simulink model "Sample_task_test"  (Simulink 8.1)
settings: Solver=ode4  SolverMode=SingleTasking  StartTime=0.0  StopTime=inf  FixedStep=0.0005  RelTol=1e-3
StartFcn:
  |  warndlg('Dexterit-E models cannot run under simulation. Please compile your model and run it from within Dexterit-E.');set_param(bdroot,'SimulationCommand','stop')
undefined symbols (not defined in the file or in its folder): slselsubs
libraries: simulink x4, General x3, KINARM_loads x2, KINARM_IO x1, KINARM_EP_loads x1, KINARM_general x1, Video x1, xpclib x1
(part 3 of 3)

== matlab function Trajectory subsystem/Create_Trajectory/get_arm_info ==
  settings: fimath=|
      | fimath(...
      | 'RoundMode', 'floor',...
      | 'OverflowMode', 'wrap',...
      | 'ProductMode', 'KeepLSB', 'ProductWordLength', 32,...
      | 'SumMode', 'KeepLSB', 'SumWordLength', 32,...
      | 'CastBeforeSum', false)
  data: position output double; task_status output double; use_dom_hand input double; kinarm_data input double; run_status input double; scaling input double; robot_enabled output double
function [position, task_status, robot_enabled]  = fcn(use_dom_hand, kinarm_data, run_status, scaling)
%
% get current hand position and robot enabled status
%
% May 2009
%

hpx_index = 23;
hpy_index = 24;
robot_disabled_index = 37;

%determine which arm to apply the load to
dominant_hand=kinarm_data(3,1);						%kinarm_data(3,1) tells which arm is the dominant arm
if use_dom_hand == 1
	feedback_arm = dominant_hand;
else
	feedback_arm = 3 - dominant_hand;
end

hpx = kinarm_data( feedback_arm, hpx_index );
hpy = kinarm_data( feedback_arm, hpy_index );
position = [hpx hpy];

if kinarm_data( feedback_arm, robot_disabled_index ) == 0;
    robot_enabled = 1;
else
    robot_enabled = 0;
end

% if the task has stopped/paused (i.e. run_status == 0) AND the torques outputs
% have scaled down to 0, then set the task_status = 0.
if run_status == 0 && scaling(feedback_arm) == 0
    task_status = 0;
else
    task_status = 1;
end

== matlab function Trajectory subsystem/KINARM_EP_Position_Controller/FF_FB_Position_Controller ==
  settings: fimath=|
      | fimath(...
      | 'RoundMode', 'floor',...
      | 'OverflowMode', 'wrap',...
      | 'ProductMode', 'KeepLSB', 'ProductWordLength', 32,...
      | 'SumMode', 'KeepLSB', 'SumWordLength', 32,...
      | 'CastBeforeSum', false)
  data: Force_FB output double; use_dom_hand input double; kinarm_data input double; setpoint_angles input double; setpoint_vel input double; setpoint_acc input double; Force_FF output double; Secondary_Encoders_Used input double; inertia_option_for_FF input double; primary_encoder_data input double; gain_choice input double; ForceOn input double
function [Force_FB, Force_FF] = fcn(use_dom_hand, kinarm_data, setpoint_angles, setpoint_vel, setpoint_acc, Secondary_Encoders_Used, inertia_option_for_FF, primary_encoder_data, gain_choice, ForceOn)
% This block supports the Embedded MATLAB subset.
% See the help menu for details. 
% set point is joint angles in global coordinates

% inertia_option_for_FF sets the options for which inertias to include for 
% the feed-forward model
%	0 - none
%	1 - KINARM robot only

% gain_choice sets the options for which proportional gains to use for the
% controller (does not affect the gains when secondary encoders are used)
%	1 - Standard Movement  == Highest stiffness. For primary encoders only, this is quite underdamped.
%	2 - Step Response == Reduced overshoot for primary encoders only, and lower stiffness.  Same as above for secondary encoders.

%{
L1_index = 1;				% L1 (m)
L2_index = 2;				% L2(m)
ORIENT_index = 6;			% 1=right	2=left
L1Ang_index = 17;			% L1 angle
L2Ang_index = 18;			% L2 Angle
L1Vel_index = 19;			% L1 angle
L2Vel_index = 20;			% L2 Angle

Force_FF = [0 0 0 0];
Force_FB = [0 0 0 0];
%}

%determine which arm to apply the load to
dominant_hand=kinarm_data(3,1);						%kinarm_data(3,1) tells which arm is the dominant arm
if use_dom_hand==1
	arm=dominant_hand;
else
	arm=3-dominant_hand;
end

%{

L1 = kinarm_data( arm, L1_index );
L2 = kinarm_data( arm, L2_index );
L1Ang = kinarm_data( arm, L1Ang_index );
L2Ang = kinarm_data( arm, L2Ang_index );
L1Vel = kinarm_data( arm, L1Vel_index );
L2Vel = kinarm_data( arm, L2Vel_index );
theta=[L1Ang; L2Ang];
thetavel=[L1Vel; L2Vel];
theta_primary = primary_encoder_data(arm, 1:2)';
thetavel_primary = primary_encoder_data(arm, 3:4)';

% Proportional Gain
if gain_choice == 1         %If the "standard movement" gain choice is selected:
    Kp = [200 0; 0 200];	%proportional gain for KINARM EP robot, primary encoders only - high stiffness
else
    Kp = [85 0; 0 85];		%proportional gain for KINARM EP robot, primary encoders only - reduced overshoot
end
Kp_1 = [0 0; 0 0];			%proportional gain for KINARM EP robot, primary encoders if used in conjunction with secondary
Kp_2 = [1 0; 0 1];		%proportional gain for KINARM EP robot, secondary encoders if used in conjunction with primary

% Derivative gain
Kv = [3.5 0; 0 3.5];		% Derivative gain for KINARM EP robot, primary encoders only				
Kv_1 = [2.5 0; 0 2.5];		% Derivative gain for KINARM EP robot, primary encoders if used in conjunction with secondary
Kv_2 = [6 0; 0 6];          % Derivative gain for KINARM EP robot, secondary encoders if used in conjunction with primary	



error = setpoint_angles - theta;
error_vel = setpoint_vel - thetavel;

error_primary = setpoint_angles - theta_primary;
error_vel_primary = setpoint_vel - thetavel_primary;

% THE FOLLOWING ARE TYPICAL VALUES FOR THE KINARM End Point robot (Rev1)
I1_prox		= 0.018;			%inertia of KINARM segment 1, kg-m^2 at shoulder
I2_5_prox	= 0.034;			%inertia of KINARM segments 2&5, kg-m^2 at elbow
I3_prox		= 0.014;			%inertia of KINARM segment 3, kg-m^2 at elbow
I4_prox		= 0.022;			%inertia of KINARM segment 4, kg-m^2 at shoulder
Im1 = 0.0047;			%inertia of motor 1, after 6x gear ratio, kg-m^2
Im2 = 0.0047;			%inertia of motor 2, after 6x gear ratio, kg-m^2
M2 = 0.62;				%mass of KINARM segment2 and 5 (kg)
M4 = 0.80;				%mass of segment 4 (kg)
L3 = 0.187;				%crank length (m)
delta = 0;				%0 degrees, angle between segments 2 and 5
x2 = 0.20;				%center of mass of segments 2+5 (m)
x4 = 0.12;				%center of mass of segment 4 (m)



theta2_1 = setpoint_angles(2) - setpoint_angles(1);
sin21 = sin(theta2_1);
cos21 = cos(theta2_1);
sin51 = sin(theta2_1 - delta);
cos51 = cos(theta2_1 - delta);

% The following equations implement the equations of motion for the KINARM robot
% For simplicity, we have ignored the off-axis components of inertia due to their
% negligible contributions
A = I1_prox + I4_prox + Im1 + M2*L1^2;
B = M2*L1*(x2*cos21) + M4*L3*(x4*cos51);
D = I2_5_prox + I3_prox + Im2 + M4*L3^2;
C = M2*L1*(x2*sin21) + M4*L3*(x4*sin51);

M = [A B; B D];	%inertial matrix
CC = [0 -C; C 0] * diag(setpoint_vel);	%coriolis and centripetal forces

if inertia_option_for_FF == 0;			%no feed-forward control
	TRQ_FF = [0; 0];
else
	TRQ_FF = M*setpoint_acc + CC*setpoint_vel;
end

if Secondary_Encoders_Used(arm) == 0
	% Only use primary encoder feedback
	TRQ_FB = Kp*error + Kv*error_vel;
else
	% Use both primary and secondary encoders - note: secondary encoder information under these conditions is contained error and error_vel
	TRQ_FB = Kp_2*error + Kv_2*error_vel + Kp_1*error_primary + Kv_1*error_vel_primary;
end

%convert torques (applied to links) to forces (applied at end-point);
A1 = -L1*sin(L1Ang);
A2 = L1*cos(L1Ang);
A3 = -L2*sin(L2Ang);
A4 = L2*cos(L2Ang);

F_FF = [A1 A2; A3 A4] \ TRQ_FF;
F_FB = [A1 A2; A3 A4] \ TRQ_FB;
%}

%%%%%%%%%%%%%%%%%%%%%%%%%%%%%%%%%%%%%%%%%%%%%%%%%%%%%%%%%%%%%%%%%%%%%%%%%%%
xPos = kinarm_data(arm,23);
yPos = kinarm_data(arm,24);
xVel = kinarm_data(arm,25);
yVel = kinarm_data(arm,26);



% FINAL FORCE CHECK
if ForceOn==1
    % Send force
    F_FB = [0; 0]; % SET WHEN EVERYTHING IS OKAY
    %F_FB = [0; 0]; % do not send force yet
else
    % No force
    F_FB = [0; 0];
end
F_FF = [0; 0];

%%%%%%%%%%%%%%%%%%%%%%%%%%%%%%%%%%%%%%%%%%%%%%%%%%%%%%%%%%%%%%%%%%%%%%%%%%%


% Flatten any bad values to 0.
if F_FF(1) ~= F_FF(1)
    F_FF(1) = 0;
end

if F_FF(2) ~= F_FF(2)
    F_FF(2) = 0;
end

if F_FB(1) ~= F_FB(1)
    F_FB(1) = 0;
end

if F_FB(2) ~= F_FB(2)
    F_FB(2) = 0;
end

%apply the forces to the correct arm 
if arm==1
	Force_FF = [F_FF' 0 0];
	Force_FB = [F_FB' 0 0];
else
	Force_FF = [0 0 F_FF'];
	Force_FB = [0 0 F_FB'];
end

== matlab function Trajectory subsystem/KINARM_EP_Position_Controller/Get_kinematics_EP/xy_to_segment_angles_EP ==
  settings: fimath=|
      | fimath(...
      | 'RoundMode', 'floor',...
      | 'OverflowMode', 'wrap',...
      | 'ProductMode', 'KeepLSB', 'ProductWordLength', 32,...
      | 'SumMode', 'KeepLSB', 'SumWordLength', 32,...
      | 'CastBeforeSum', false)
  data: use_dom_hand input double; kinarm_data input double; u input double; SEGMENT_ANG output double; robot_calib input double
function SEGMENT_ANG  = fcn(use_dom_hand, kinarm_data, u, robot_calib)

% This function converts an endpoint finger-tip position or local joint angle (shoulder, elbow) 
% to (L1Ang, L2Ang) angles for a KINARM robot where L1Ang and L2Ang are the global angles of L1 and L2  
% Note: these equations were taken from a source which defined theta1 as the global angle of L1 (i.e. theta1 = L1Ang
% and L2_L1Ang = local angle of L2 WRT L1 (but always in a R.H. coordinate frame).  So L2_L1Ang = L2Ang - L1Ang.
% Also note that we need to correct for L2_ptr

% angles_or_XY sets the options for which coordinate system to use
%	1 - (x, y) coordinates
%	2 - local coordinate joint angles (shoulder, elbow)

% NEED TO GET SHOULDER AND ELBOW ANGLE OFFSETS FROM CALIBRATION WHEN THESE BECOME AVAILABLE.
% For the KINARM End-Point robot I have assumed certain values, which will hold unless the robot
% is mounted at an angle relative to global.
% Need to decide how to deal with this for the Exoskeleton lab.

L1_index = 1;				% L1 (m)
L2_index = 2;				% L2(m)
L2ptr_index = 3;			% L2ptr(m)
SHO_ORIGIN_X_index = 4;		% shoulder origin, x position
SHO_ORIGIN_Y_index = 5;		% shoulder origin, y position
ORIENT_index = 6;			% 1=right	2=left


%determine which arm to apply the load to
dominant_hand=kinarm_data(3,1);						%kinarm_data(3,1) tells which arm is the dominant arm
if use_dom_hand==1
	arm=dominant_hand;
else
	arm=3-dominant_hand;
end

ORIENTATION = kinarm_data( arm, ORIENT_index);

% To be consistent with the Exoskeleton, the shoulder and elbow angles are stored in a 
% 'local' coordinate frame from the robot's perspective.  The right End-Point robot is 
% constructed the same a left KINARM Exoskeleton and vice-versa.  So the 'local' coordinate
% frame for a R.H. KINARM EP robot is actually a left-handed coordinate frame.
Sho_offset = robot_calib(1, arm);		% value stored in calibration in a 'local' coordinate frame.

position=[0,0];	%initialization
if length(u)==2	%input is assumed to be (x,y) position, global coordinates, (m)
    if size(u,1) == 1;
        position=u;
    else
        position=u';
    end
else			%input is assumed to be a VCODE
    position(1)=u(3);
    position(2)=u(4);
end


% calculate theta from (x,y)
L1 = kinarm_data( arm, L1_index );
L2 = kinarm_data( arm, L2_index );
L2ptr = kinarm_data( arm, L2ptr_index );
SHO_ORIGIN_X = kinarm_data( arm, SHO_ORIGIN_X_index );
SHO_ORIGIN_Y = kinarm_data( arm, SHO_ORIGIN_Y_index );

x = position(1) - SHO_ORIGIN_X;
y = position(2) - SHO_ORIGIN_Y;

L2_temp = sqrt(L2^2 + L2ptr^2);
L2_ptr_angle_shift = atan2(L2ptr, L2);			%

% The following calculation assumes that the (local) elbow angle is 
% never less than 0 (i.e. L2_L1Ang > 0 for right-handed Exoskeleton, or LEFT-HANDED End-Point, and 
% L2_L1Ang < 0 for  left-handed Exoskelton or RIGHT-HANDED End-Point).  These are always true if L2ptr > 0.  
% If L2ptr < 0, then two solutions exist, however, the one with (local) 
% elbow_angle > 0 is chosen.  
% In addition, temp is limited to +-1 to avoid an error using acos.  
% Originally this was simple clipping, but the infinite slope at acos(1)
% created instability problems, so tanh(temp + temp^3/3...) was added to 
% smooth out the transition.  The difference in angle is < 1 degree with 
% elbow angle > 30 degrees.  As the elbow extends further, the 'error' 
% is <20 degrees when full extension should theoretically happen.  For 
% L1 = 0.3m and L2 = 0.4m, the end-point error with an input point
% that in theory requires full extension is <1cm.  This end-point error
% is < 1mm when the desired endpoint is >66cm out.
% Note: tanh(temp + temp^3/3...) provides a sharper transition than 
% tanh(temp), which in turn provides a shaper one than atan(temp)
% The more terms in the tanh(temp...) series, the greater the cutoff
temp = (x^2 + y^2 - L1^2 - L2_temp^2) / (2*L1*L2_temp);
% 	temp = sign(temp) * min(abs(temp), 1);          %Not used to avoid infinite slope issue for subsequent acos
temp = tanh(temp + temp^3/3 + temp^5/5 + temp^7/7 + temp^9/9 + temp^11/11);
L2_L1Ang = acos( temp );

% if ORIENTATION == 2 %left-handed KINARM Exoskeleton 
if ORIENTATION == 1 %right-handed KINARM End-Point robot
    L2_L1Ang = -L2_L1Ang;
    L2_ptr_angle_shift = -L2_ptr_angle_shift;
end
sint = sin(L2_L1Ang);
cost = cos(L2_L1Ang);
L1Ang = atan2( ( -x*L2_temp*sint + y *(L1 + L2_temp*cost) ) , ( y*L2_temp*sint + x *(L1 + L2_temp*cost) ) );

% Likewise, there are multiple solutions for the inverse kinematics for 
% L1Ang as well. We know (based on possible arm configurations) which is 
% the correct solution for right-handed versus left-handed KINARMs.
% Sho_offset is in local coordinates.  It is translated to global as  
% L1_offset.  For "left" robots (i.e. left Exo and right EP), 
% L1Ang = -ShoAng + pi.  
% For the KINARM End-Point robot, working from the calibration 
% position (i.e. when L1Ang = L1_Offset), we know that the L1 link cannot 
% point directly backwards into the K-box.  Which for the left KINARM EP is 
% a rotation of -3/4pi or +5/4pi and for the right it is -5/4pi or +3/4pi.

if ORIENTATION == 2 
	% left-handed KINARM End_point
    L1_offset = Sho_offset;
    if L1Ang < (L1_offset - 3/4*pi) 
        L1Ang = L1Ang + 2*pi;
    elseif L1Ang > (L1_offset + 5/4*pi)
        L1Ang = L1Ang - 2*pi;
    end
else
    L1_offset = -Sho_offset + pi;
    if L1Ang < (L1_offset - 5/4*pi) 
        L1Ang = L1Ang + 2*pi;
    elseif L1Ang > (L1_offset + 3/4*pi)
        L1Ang = L1Ang - 2*pi;
    end

end

L2Ang = L1Ang + L2_L1Ang - L2_ptr_angle_shift;

SEGMENT_ANG = [L1Ang; L2Ang];

== matlab function Draw_Hand_Endpoint/MATLAB Function ==
  data: target input double; VCODE output double; state_in input double; target_type input double; opacity_in input double; target_display input double; x_index input double; y_index input double; num_states input double; stateindices input double; target_labels input double; KINData input double; CursorOpacity input double
function VCODE = fcn(target, state_in, target_type, opacity_in, target_display, x_index, y_index, num_states, stateindices, target_labels, KINData, CursorOpacity)

% stateindices should follow this order (depending on target-type):
% 1: length of tool (m)
% 2: stroke colour
% 3: stroke width
% 4: major radius / radius / start point (line)
% 5: minor radius / end point (line)
% 6: orientation angle



% VCODEs are length 70. All units in a VCODE should be SI, e.g. (m) and (rad). Elements in a VCODE are defined as follows:
%
% For all target types:
%  1: target type
%       1 - circle
%       2 - ellipse
%       3 - rectangle
%       4 - line
%       5 - triangle
%       11 - circle with label
%       12 - ellipse with label
%       13 - rectangle with label
%       14 - line with label
%       15 - triangle with label
%  2: target on/off status and target display (which display target will appear on)
%		0 - off
%		1 - on, appearing on both subject and operator displays
%       2 - on, appearing on subject display only
%       3 - on, appearing on operator display only
%  3: x position (m)
%  4: y position (m)
%  5: fill colour (RRGGBB) or texture index
%  6: stroke colour (RRGGBB) or texture index
%  7: stroke width
%  8: reserved for target background ID
%  9: opacity
%
% For circles:
%  10: radius (m)
%
% For ellipses:
%  10: major radius (m)
%  11: minor radius (m)
%  12: orientation of major axis (rad)
%
% For rectangles:
%  10: length (m)
%  11: height (m)
%  12: orientation (rad) (relative to x, y already shown)
%
% For lines:
%  10: endpoint x-axis coordinate relative to start point (m)
%  11: endpoint y-axis coordinate relative to start point (m)
%
% For triangles:
%  10: length (m)
%  11: height (m)
%  12: offset of peak from midpoint of length (m)
%  13: orientation (rad)
%
% For all labelled target types:
%  14: reserved
%  15-64: label characters (indexes in ISO 8859-1 character set)
%  65: label colour (0xRRGGBB), opacity is set by the vcode's opacity (9).
%  66: label height (m)
%  67: reserved
%  68: reserved
%  69: reserved
%  70: reserved

num_targets = size(target, 1);

% NOTE: we assume that the STATE and/or OPACITY inputs are vectors. 

% If the length of the input STATE is not the same as the number of targets then make STATE a column vector of the same length as 
% the TARGET input, using the first STATE (i.e. all targets get the same state) 
if num_targets == length(state_in)
	state = reshape(state_in, num_targets, 1);
else
	state = state_in(1) * ones(num_targets, 1);
end


% If the length of the input OPACITY is not the same as the number of targets then make OPACITY a column vector of the same length as
% the TARGET input, using the first OPACITY (i.e. all targets get the same opacity) 
if num_targets == length(opacity_in)
	opacity = reshape(opacity_in, num_targets, 1);
else
	opacity = opacity_in(1) * ones(num_targets, 1);
end


% Clamping the opacity to [0, 100].
opacity = min(opacity, 100);
opacity = max(opacity, 0);

VCODE = zeros(num_targets, 70);

% Set the target type. Targets with labels have type codes 10 greater than their unlabelled counterparts.
VCODE(:, 1) = target_type + 10;

% Set the hand position.
VCODE(:, 3) = KINData(1,23);  % x position (m)
VCODE(:, 4) = KINData(1,24);  % y position (m)

for ii = 1:num_targets
	% Set the target on/off state. If the state input is 0, the target is off. Users of the VCODE should respect this
	% as an indication that the rest of the VCODE will be uninitialized.
	if (state(ii) <= 0) || (state(ii) > num_states)
		VCODE(ii, 2) = 0;  % target is off
	else
		VCODE(ii, 2) = target_display;  % Default is that target is on; target displays as specified by block mask
	end

	fill_colour_col = stateindices(state(ii), 1);
	stroke_colour_col = stateindices(state(ii), 2);
	stroke_width_col = stateindices(state(ii), 3);
	
	% Set the fill colour. Fill colour currently comes from the GUI in RRRGGGBBB format.
	if fill_colour_col == 0
		VCODE(ii, 5) = -2^31;
	elseif target(fill_colour_col) < 0
		VCODE(ii, 5) = target(ii, fill_colour_col);
	else
		VCODE(ii, 5) = colourshift(target(ii, fill_colour_col));
	end
	
	% Set the stroke colour. Stroke colour currently comes from the GUI in RRRGGGBBB format.
	if stroke_colour_col == 0
		VCODE(ii, 6) = -2^31;
	elseif target(stroke_colour_col) < 0
		VCODE(ii, 6) = target(ii, stroke_colour_col);
	else
		VCODE(ii, 6) = colourshift( target(ii, stroke_colour_col) );
	end

	% Set the stroke width. if target table index for stroke width is zero, then the stroke width is undefined
	if stroke_width_col == 0
		VCODE(ii, 7) = 0;                   % if stroke width column is 0, then stroke width is 0
	elseif stroke_width_col < 0
		VCODE(ii, 7) = 0.001;               % if stroke width column is -ve, then a 1mm default is chosen
	else
		VCODE(ii, 7) = target(ii, stroke_width_col) * 0.01;  % if stroke width column is +ve, convert width from (cm) in target table to (m)
	end

	% Set the opacity value
	VCODE(ii, 9) = CursorOpacity;

	% Set attributes specific to each target type. In the process, note the first state vector column used for label information.
	label_index = 1;

	% Set attributes specific to each target type.
	if target_type == 1

		% Handle circle target:
		radius_col = stateindices(state(ii), 4);
		VCODE(ii, 10)=target(ii, radius_col);  % radius (convert from (cm) in target table to (m))
	    label_index = 5;

	elseif target_type == 2 || target_type == 3

	    % Handle ellipse or rectangle target:
		major_col = stateindices(state(ii), 4);
		minor_col = stateindices(state(ii), 5);
		orientation_col = stateindices(state(ii), 6);
		
		VCODE(ii, 10) = target(ii, major_col) * 0.01;  % major radius (convert from (cm) in target table to (m))
		VCODE(ii, 11) = target(ii, minor_col) * 0.01;  % minor radius (convert from (cm) in target table to (m))
		if orientation_col == 0
			VCODE(ii, 12) = 0;  % if orientation column is 0, set orientation to 0 rad
		else
			VCODE(ii, 12) = mod(target(ii, orientation_col), 360) * pi / 180.0;  % orientation (convert from (degrees) in target table to (rad))
		end
	    label_index = 7;
	
	elseif target_type == 4

		% Handle line target:
		%xendpoint_col = stateindices(state(ii), 4);
		%yendpoint_col = stateindices(state(ii), 5);
		VCODE(ii, 10) = 0;  % line endpoint in x axis, relative to start (m)
		VCODE(ii, 11) = stateindices(state(ii), 1);  % line endpoint in y axis, relative to start (taken from Target Table)
	    label_index = 6;

	elseif target_type == 5

		% Handle triangle target:
		length_col = stateindices(state(ii), 4);
		height_col = stateindices(state(ii), 5);
		offset_col = stateindices(state(ii), 6);
		orientation_col = stateindices(state(ii), 7);

		VCODE(ii, 10) = target(ii, length_col) * 0.01;  % length (convert from (cm) in target table to (m))

		% If the height column is set to 0 then the triangle is automatically made equilateral, with the base length used as length
		% for all sides. If the height column is non-zero, separate values for height and peak offset are taken from the target table.
		if height_col == 0
			VCODE(ii, 11) = sin(pi / 3.0) * VCODE(ii, 10);  % height for equilateral triangle
			VCODE(ii, 12) = 0;                          % peak offset for equilateral triangle
		else
			VCODE(ii, 11) = target(ii, height_col) * 0.01;  % height (convert from (cm) in target table to (m))
			VCODE(ii, 12) = target(ii, offset_col) * 0.01;  % peak offset (convert from (cm) in target table to (m))
		end

		if orientation_col == 0
			VCODE(ii, 13) = 0;  % if orientation column is 0, set orientation to 0 rad
		else
			VCODE(ii, 13) = mod(target(ii, orientation_col), 360) * pi / 180.0;  % orientation (convert from (degrees) in target table to (rad))
		end
	    label_index = 8;
		
	end
	
	% Copy the label characters to the VCODE.
	for jj = 1:50
		VCODE(ii, jj + 14) = target_labels( target( ii, stateindices(state(ii), label_index) ), jj );
	end

	% Set the label colour. Like other colours, label colour comes from the GUI in RRRGGGBBB format and is converted to a 32-bit
	% 0xRRGGBB value here. If the target column table index for the colour is 0, the label is transparent.
	if stateindices(state(ii), label_index + 1) == 0
		VCODE(ii, 65) = -2^31;
	elseif target( ii, stateindices(state(ii), label_index + 1) ) < 0
		VCODE(ii, 65) = target( ii, stateindices(state(ii), label_index + 1) );
	else
		VCODE(ii, 65) = colourshift( target( ii, stateindices(state(ii), label_index + 1) ) );
	end

	% Set the label height. Label height is converted from (cm) in the target table to (m).
	VCODE(ii, 66) = target( ii, stateindices(state, label_index + 2) ) * 0.01;


	
end

% The colourshift function converts an "RRRGGGBBB" colour value to RRGBB (as an uint32).
function RRGGBBAA = colourshift(RRRGGGBBB)

%this is "no fill"
if RRRGGGBBB == 1000000000
    RRGGBBAA = cast(16777216, 'uint32'); %hex 0x1000000
    return; 
end

blue = cast(mod(RRRGGGBBB, 1000), 'uint32');
green = cast(mod(RRRGGGBBB - blue, 1000000) / 1000, 'uint32');
red = cast((RRRGGGBBB - (green * 1000) - blue) / 1000000, 'uint32');

RRGGBBAA = bitshift(red, 16) + bitshift(green, 8) + blue;

== matlab function Parameter_columns/MATLAB Function ==
  data: target input double; VCODE output double; state_in input double; target_type input double; opacity_in input double; target_display input double; x_index input double; y_index input double; num_states input double; stateindices input double; target_labels input double
function VCODE = fcn(target, state_in, target_type, opacity_in, target_display, x_index, y_index, num_states, stateindices, target_labels)

VCODE = zeros(1,70);
% SIMPLY ASSIGN TOOL LENGTH AND WIDTH TO OUTPUT, NOT REAL VCODE!!
VCODE(1,1) = target(1,stateindices(1,1)); % tool width (m)
VCODE(1,2) = target(1,stateindices(1,2)); % tool length (m)
VCODE(1,3) = target(1,stateindices(1,3)); % frame inner width (m)
VCODE(1,4) = target(1,stateindices(1,4)); % frame outer width (m)
VCODE(1,5) = target(1,stateindices(1,5)); % force on?
VCODE(1,6) = target(1,stateindices(1,6)); % start radius (m)
VCODE(1,7) = target(1,stateindices(1,7)); % end radius (m)
%{
% stateindices should follow this order (depending on target-type):
% 1: fill colour
% 2: stroke colour
% 3: stroke width
% 4: major radius / radius / start point (line)
% 5: minor radius / end point (line)
% 6: orientation angle



% VCODEs are length 70. All units in a VCODE should be SI, e.g. (m) and (rad). Elements in a VCODE are defined as follows:
%
% For all target types:
%  1: target type
%       1 - circle
%       2 - ellipse
%       3 - rectangle
%       4 - line
%       5 - triangle
%       11 - circle with label
%       12 - ellipse with label
%       13 - rectangle with label
%       14 - line with label
%       15 - triangle with label
%  2: target on/off status and target display (which display target will appear on)
%		0 - off
%		1 - on, appearing on both subject and operator displays
%       2 - on, appearing on subject display only
%       3 - on, appearing on operator display only
%  3: x position (m)
%  4: y position (m)
%  5: fill colour (RRGGBB) or texture index
%  6: stroke colour (RRGGBB) or texture index
%  7: stroke width
%  8: reserved for target background ID
%  9: opacity
%
% For circles:
%  10: radius (m)
%
% For ellipses:
%  10: major radius (m)
%  11: minor radius (m)
%  12: orientation of major axis (rad)
%
% For rectangles:
%  10: length (m)
%  11: height (m)
%  12: orientation (rad) (relative to x, y already shown)
%
% For lines:
%  10: endpoint x-axis coordinate relative to start point (m)
%  11: endpoint y-axis coordinate relative to start point (m)
%
% For triangles:
%  10: length (m)
%  11: height (m)
%  12: offset of peak from midpoint of length (m)
%  13: orientation (rad)
%
% For all labelled target types:
%  14: reserved
%  15-64: label characters (indexes in ISO 8859-1 character set)
%  65: label colour (0xRRGGBB), opacity is set by the vcode's opacity (9).
%  66: label height (m)
%  67: reserved
%  68: reserved
%  69: reserved
%  70: reserved

num_targets = size(target, 1);

% NOTE: we assume that the STATE and/or OPACITY inputs are vectors. 

% If the length of the input STATE is not the same as the number of targets then make STATE a column vector of the same length as 
% the TARGET input, using the first STATE (i.e. all targets get the same state) 
if num_targets == length(state_in)
	state = reshape(state_in, num_targets, 1);
else
	state = state_in(1) * ones(num_targets, 1);
end


% If the length of the input OPACITY is not the same as the number of targets then make OPACITY a column vector of the same length as
% the TARGET input, using the first OPACITY (i.e. all targets get the same opacity) 
if num_targets == length(opacity_in)
	opacity = reshape(opacity_in, num_targets, 1);
else
	opacity = opacity_in(1) * ones(num_targets, 1);
end


% Clamping the opacity to [0, 100].
opacity = min(opacity, 100);
opacity = max(opacity, 0);

VCODE = zeros(num_targets, 70);

% Set the target type. Targets with labels have type codes 10 greater than their unlabelled counterparts.
VCODE(:, 1) = target_type + 10;

% Set the target position.
VCODE(:, 3) = target(:, x_index) * 0.01;  % x position (convert from (cm) in target table to (m))
VCODE(:, 4) = target(:, y_index) * 0.01;  % y position (convert from (cm) in target table to (m))

for ii = 1:num_targets
	% Set the target on/off state. If the state input is 0, the target is off. Users of the VCODE should respect this
	% as an indication that the rest of the VCODE will be uninitialized.
	if (state(ii) <= 0) || (state(ii) > num_states)
		VCODE(ii, 2) = 0;  % target is off
	else
		VCODE(ii, 2) = target_display;  % Default is that target is on; target displays as specified by block mask
	end

	fill_colour_col = stateindices(state(ii), 1);
	stroke_colour_col = stateindices(state(ii), 2);
	stroke_width_col = stateindices(state(ii), 3);
	
	% Set the fill colour. Fill colour currently comes from the GUI in RRRGGGBBB format.
	if fill_colour_col == 0
		VCODE(ii, 5) = -2^31;
	elseif target(fill_colour_col) < 0
		VCODE(ii, 5) = target(ii, fill_colour_col);
	else
		VCODE(ii, 5) = colourshift(target(ii, fill_colour_col));
	end
	
	% Set the stroke colour. Stroke colour currently comes from the GUI in RRRGGGBBB format.
	if stroke_colour_col == 0
		VCODE(ii, 6) = -2^31;
	elseif target(stroke_colour_col) < 0
		VCODE(ii, 6) = target(ii, stroke_colour_col);
	else
		VCODE(ii, 6) = colourshift( target(ii, stroke_colour_col) );
	end

	% Set the stroke width. if target table index for stroke width is zero, then the stroke width is undefined
	if stroke_width_col == 0
		VCODE(ii, 7) = 0;                   % if stroke width column is 0, then stroke width is 0
	elseif stroke_width_col < 0
		VCODE(ii, 7) = 0.001;               % if stroke width column is -ve, then a 1mm default is chosen
	else
		VCODE(ii, 7) = target(ii, stroke_width_col) * 0.01;  % if stroke width column is +ve, convert width from (cm) in target table to (m)
	end

	% Set the opacity value
	VCODE(ii, 9) = opacity(ii);

	% Set attributes specific to each target type. In the process, note the first state vector column used for label information.
	label_index = 1;

	% Set attributes specific to each target type.
	if target_type == 1

		% Handle circle target:
		radius_col = stateindices(state(ii), 4);
		VCODE(ii, 10)=target(ii, radius_col) * 0.01;  % radius (convert from (cm) in target table to (m))
	    label_index = 5;

	elseif target_type == 2 || target_type == 3

	    % Handle ellipse or rectangle target:
		major_col = stateindices(state(ii), 4);
		minor_col = stateindices(state(ii), 5);
		orientation_col = stateindices(state(ii), 6);
		
		VCODE(ii, 10) = target(ii, major_col) * 0.01;  % major radius (convert from (cm) in target table to (m))
		VCODE(ii, 11) = target(ii, minor_col) * 0.01;  % minor radius (convert from (cm) in target table to (m))
		if orientation_col == 0
			VCODE(ii, 12) = 0;  % if orientation column is 0, set orientation to 0 rad
		else
			VCODE(ii, 12) = mod(target(ii, orientation_col), 360) * pi / 180.0;  % orientation (convert from (degrees) in target table to (rad))
		end
	    label_index = 7;
	
	elseif target_type == 4

		% Handle line target:
		xendpoint_col = stateindices(state(ii), 4);
		yendpoint_col = stateindices(state(ii), 5);
		VCODE(ii, 10) = target(ii, xendpoint_col) * 0.01;  % line endpoint in x axis, relative to start (convert from (cm) in target table to (m))
		VCODE(ii, 11) = target(ii, yendpoint_col) * 0.01;  % line endpoint in y axis, relative to start (convert from (cm) in target table to (m))
	    label_index = 6;

	elseif target_type == 5

		% Handle triangle target:
		length_col = stateindices(state(ii), 4);
		height_col = stateindices(state(ii), 5);
		offset_col = stateindices(state(ii), 6);
		orientation_col = stateindices(state(ii), 7);

		VCODE(ii, 10) = target(ii, length_col) * 0.01;  % length (convert from (cm) in target table to (m))

		% If the height column is set to 0 then the triangle is automatically made equilateral, with the base length used as length
		% for all sides. If the height column is non-zero, separate values for height and peak offset are taken from the target table.
		if height_col == 0
			VCODE(ii, 11) = sin(pi / 3.0) * VCODE(ii, 10);  % height for equilateral triangle
			VCODE(ii, 12) = 0;                          % peak offset for equilateral triangle
		else
			VCODE(ii, 11) = target(ii, height_col) * 0.01;  % height (convert from (cm) in target table to (m))
			VCODE(ii, 12) = target(ii, offset_col) * 0.01;  % peak offset (convert from (cm) in target table to (m))
		end

		if orientation_col == 0
			VCODE(ii, 13) = 0;  % if orientation column is 0, set orientation to 0 rad
		else
			VCODE(ii, 13) = mod(target(ii, orientation_col), 360) * pi / 180.0;  % orientation (convert from (degrees) in target table to (rad))
		end
	    label_index = 8;
		
	end
	
	% Copy the label characters to the VCODE.
	for jj = 1:50
		VCODE(ii, jj + 14) = target_labels( target( ii, stateindices(state(ii), label_index) ), jj );
	end

	% Set the label colour. Like other colours, label colour comes from the GUI in RRRGGGBBB format and is converted to a 32-bit
	% 0xRRGGBB value here. If the target column table index for the colour is 0, the label is transparent.
	if stateindices(state(ii), label_index + 1) == 0
		VCODE(ii, 65) = -2^31;
	elseif target( ii, stateindices(state(ii), label_index + 1) ) < 0
		VCODE(ii, 65) = target( ii, stateindices(state(ii), label_index + 1) );
	else
		VCODE(ii, 65) = colourshift( target( ii, stateindices(state(ii), label_index + 1) ) );
	end

	% Set the label height. Label height is converted from (cm) in the target table to (m).
	VCODE(ii, 66) = target( ii, stateindices(state, label_index + 2) ) * 0.01;


	
end

% The colourshift function converts an "RRRGGGBBB" colour value to RRGBB (as an uint32).
function RRGGBBAA = colourshift(RRRGGGBBB)

%this is "no fill"
if RRRGGGBBB == 1000000000
    RRGGBBAA = cast(16777216, 'uint32'); %hex 0x1000000
    return; 
end

blue = cast(mod(RRRGGGBBB, 1000), 'uint32');
green = cast(mod(RRRGGGBBB - blue, 1000000) / 1000, 'uint32');
red = cast((RRRGGGBBB - (green * 1000) - blue) / 1000000, 'uint32');

RRGGBBAA = bitshift(red, 16) + bitshift(green, 8) + blue;
%}

== matlab function Hand_at_start ==
  data: HandAtStart output double; SET_EXP_PARAMS1 input double; KINdata input double; xStart output double; yStart output double; xEnd output double; yEnd output double; HandVelX output double; HandVelY output double
function [HandAtStart,xStart,yStart,xEnd,yEnd,HandVelX,HandVelY] = Hand_at_start(SET_EXP_PARAMS1, KINdata)

% Position of robot during whole task
xStart = SET_EXP_PARAMS1(1);
yStart = SET_EXP_PARAMS1(2);

xEnd = SET_EXP_PARAMS1(3);
yEnd = SET_EXP_PARAMS1(4);

% Start and end radius of movement
StartRadius = SET_EXP_PARAMS1(5);

% Check to see if hand or tool endpoint is in target
HandPosX = KINdata(1,23);
HandPosY = KINdata(1,24);
HandVelX = KINdata(1,25);
HandVelY = KINdata(1,26);

% Is hand inside (xInit,yInit)?
HandAtStart = double(sqrt((HandPosX-xStart)^2+(HandPosY-yStart)^2)<StartRadius);

== matlab function Draw_Start_Circle/MATLAB Function ==
  data: target input double; VCODE output double; state_in input double; target_type input double; opacity_in input double; target_display input double; x_index input double; y_index input double; num_states input double; stateindices input double; target_labels input double; KINData input double; xStart input double; yStart input double; trial_state input double
function VCODE = fcn(target, state_in, target_type, opacity_in, target_display, x_index, y_index, num_states, stateindices, target_labels, KINData, xStart, yStart, trial_state)

% stateindices should follow this order (depending on target-type):
% 1: fill colour
% 2: stroke colour
% 3: stroke width
% 4: major radius / radius / start point (line)
% 5: minor radius / end point (line)
% 6: orientation angle



% VCODEs are length 70. All units in a VCODE should be SI, e.g. (m) and (rad). Elements in a VCODE are defined as follows:
%
% For all target types:
%  1: target type
%       1 - circle
%       2 - ellipse
%       3 - rectangle
%       4 - line
%       5 - triangle
%       11 - circle with label
%       12 - ellipse with label
%       13 - rectangle with label
%       14 - line with label
%       15 - triangle with label
%  2: target on/off status and target display (which display target will appear on)
%		0 - off
%		1 - on, appearing on both subject and operator displays
%       2 - on, appearing on subject display only
%       3 - on, appearing on operator display only
%  3: x position (m)
%  4: y position (m)
%  5: fill colour (RRGGBB) or texture index
%  6: stroke colour (RRGGBB) or texture index
%  7: stroke width
%  8: reserved for target background ID
%  9: opacity
%
% For circles:
%  10: radius (m)
%
% For ellipses:
%  10: major radius (m)
%  11: minor radius (m)
%  12: orientation of major axis (rad)
%
% For rectangles:
%  10: length (m)
%  11: height (m)
%  12: orientation (rad) (relative to x, y already shown)
%
% For lines:
%  10: endpoint x-axis coordinate relative to start point (m)
%  11: endpoint y-axis coordinate relative to start point (m)
%
% For triangles:
%  10: length (m)
%  11: height (m)
%  12: offset of peak from midpoint of length (m)
%  13: orientation (rad)
%
% For all labelled target types:
%  14: reserved
%  15-64: label characters (indexes in ISO 8859-1 character set)
%  65: label colour (0xRRGGBB), opacity is set by the vcode's opacity (9).
%  66: label height (m)
%  67: reserved
%  68: reserved
%  69: reserved
%  70: reserved

num_targets = size(target, 1);

% NOTE: we assume that the STATE and/or OPACITY inputs are vectors. 

% If the length of the input STATE is not the same as the number of targets then make STATE a column vector of the same length as 
% the TARGET input, using the first STATE (i.e. all targets get the same state)
if num_targets == length(state_in)
	state = reshape(state_in, num_targets, 1);
else
	state = state_in(1) * ones(num_targets, 1);
end


% If the length of the input OPACITY is not the same as the number of targets then make OPACITY a column vector of the same length as
% the TARGET input, using the first OPACITY (i.e. all targets get the same opacity)
if num_targets == length(opacity_in)
	opacity = reshape(opacity_in, num_targets, 1);
else
	opacity = opacity_in(1) * ones(num_targets, 1);
end


% Clamping the opacity to [0, 100].
opacity = min(opacity, 100);
opacity = max(opacity, 0);

VCODE = zeros(num_targets, 70);

% Set the target type. Targets with labels have type codes 10 greater than their unlabelled counterparts.
VCODE(:, 1) = target_type + 10;

% Set the hand position.
VCODE(:, 3) = xStart;  % x position (m)
VCODE(:, 4) = yStart;  % y position (m)

for ii = 1:num_targets
	% Set the target on/off state. If the state input is 0, the target is off. Users of the VCODE should respect this
	% as an indication that the rest of the VCODE will be uninitialized.
	if (state(ii) <= 0) || (state(ii) > num_states)
		VCODE(ii, 2) = 0;  % target is off
	else
		VCODE(ii, 2) = target_display;  % Default is that target is on; target displays as specified by block mask
	end

	fill_colour_col = stateindices(state(ii), 1);
	stroke_colour_col = stateindices(state(ii), 2);
	stroke_width_col = stateindices(state(ii), 3);
	
	% Set the fill colour. Fill colour currently comes from the GUI in RRRGGGBBB format.
	%{
    if fill_colour_col == 0
		VCODE(ii, 5) = -2^31;
	elseif target(fill_colour_col) < 0
		VCODE(ii, 5) = target(ii, fill_colour_col);
	else
		VCODE(ii, 5) = colourshift(target(ii, fill_colour_col));
    end
    %}
    VCODE(ii,5) = colourshift(1000000000);
	
	% Set the stroke colour. Stroke colour currently comes from the GUI in RRRGGGBBB format.
	if stroke_colour_col == 0
		VCODE(ii, 6) = -2^31;
	elseif target(stroke_colour_col) < 0
		VCODE(ii, 6) = target(ii, stroke_colour_col);
	else
		VCODE(ii, 6) = colourshift( target(ii, stroke_colour_col) );
    end

	% Set the stroke width. if target table index for stroke width is zero, then the stroke width is undefined
	if stroke_width_col == 0
		VCODE(ii, 7) = 0;                   % if stroke width column is 0, then stroke width is 0
	elseif stroke_width_col < 0
		VCODE(ii, 7) = 0.001;               % if stroke width column is -ve, then a 1mm default is chosen
	else
		VCODE(ii, 7) = target(ii, stroke_width_col) * 0.01 * 3;  % if stroke width column is +ve, convert width from (cm) in target table to (m)
    end

	% Set the opacity value
	VCODE(ii, 9) = opacity(ii);

	% Set attributes specific to each target type. In the process, note the first state vector column used for label information.
	label_index = 1;

	% Set attributes specific to each target type.
	if target_type == 1

		% Handle circle target:
		radius_col = stateindices(state(ii), 4);
		VCODE(ii, 10)=target(ii, radius_col);  % radius (in m)
	    label_index = 5;

	elseif target_type == 2 || target_type == 3

	    % Handle ellipse or rectangle target:
		major_col = stateindices(state(ii), 4);
		minor_col = stateindices(state(ii), 5);
		orientation_col = stateindices(state(ii), 6);
		
		VCODE(ii, 10) = target(ii, major_col) * 0.01;  % major radius (convert from (cm) in target table to (m))
		VCODE(ii, 11) = target(ii, minor_col) * 0.01;  % minor radius (convert from (cm) in target table to (m))
		if orientation_col == 0
			VCODE(ii, 12) = 0;  % if orientation column is 0, set orientation to 0 rad
		else
			VCODE(ii, 12) = mod(target(ii, orientation_col), 360) * pi / 180.0;  % orientation (convert from (degrees) in target table to (rad))
		end
	    label_index = 7;
	
	elseif target_type == 4

		% Handle line target:
		%xendpoint_col = stateindices(state(ii), 4);
		%yendpoint_col = stateindices(state(ii), 5);
		VCODE(ii, 10) = 0;  % line endpoint in x axis, relative to start (m)
		VCODE(ii, 11) = stateindices(state(ii), 1);  % line endpoint in y axis, relative to start (taken from Target Table)
	    label_index = 6;

	elseif target_type == 5

		% Handle triangle target:
		length_col = stateindices(state(ii), 4);
		height_col = stateindices(state(ii), 5);
		offset_col = stateindices(state(ii), 6);
		orientation_col = stateindices(state(ii), 7);

		VCODE(ii, 10) = target(ii, length_col) * 0.01;  % length (convert from (cm) in target table to (m))

		% If the height column is set to 0 then the triangle is automatically made equilateral, with the base length used as length
		% for all sides. If the height column is non-zero, separate values for height and peak offset are taken from the target table.
		if height_col == 0
			VCODE(ii, 11) = sin(pi / 3.0) * VCODE(ii, 10);  % height for equilateral triangle
			VCODE(ii, 12) = 0;                          % peak offset for equilateral triangle
		else
			VCODE(ii, 11) = target(ii, height_col) * 0.01;  % height (convert from (cm) in target table to (m))
			VCODE(ii, 12) = target(ii, offset_col) * 0.01;  % peak offset (convert from (cm) in target table to (m))
		end

		if orientation_col == 0
			VCODE(ii, 13) = 0;  % if orientation column is 0, set orientation to 0 rad
		else
			VCODE(ii, 13) = mod(target(ii, orientation_col), 360) * pi / 180.0;  % orientation (convert from (degrees) in target table to (rad))
		end
	    label_index = 8;
		
	end
	
	% Copy the label characters to the VCODE.
	for jj = 1:50
		VCODE(ii, jj + 14) = target_labels( target( ii, stateindices(state(ii), label_index) ), jj );
	end

	% Set the label colour. Like other colours, label colour comes from the GUI in RRRGGGBBB format and is converted to a 32-bit
	% 0xRRGGBB value here. If the target column table index for the colour is 0, the label is transparent.
	if stateindices(state(ii), label_index + 1) == 0
		VCODE(ii, 65) = -2^31;
	elseif target( ii, stateindices(state(ii), label_index + 1) ) < 0
		VCODE(ii, 65) = target( ii, stateindices(state(ii), label_index + 1) );
	else
		VCODE(ii, 65) = colourshift( target( ii, stateindices(state(ii), label_index + 1) ) );
	end

	% Set the label height. Label height is converted from (cm) in the target table to (m).
	VCODE(ii, 66) = target( ii, stateindices(state, label_index + 2) ) * 0.01;


	
end

% The colourshift function converts an "RRRGGGBBB" colour value to RRGBB (as an uint32).
function RRGGBBAA = colourshift(RRRGGGBBB)

%this is "no fill"
if RRRGGGBBB == 1000000000
    RRGGBBAA = cast(16777216, 'uint32'); %hex 0x1000000
    return; 
end

blue = cast(mod(RRRGGGBBB, 1000), 'uint32');
green = cast(mod(RRRGGGBBB - blue, 1000000) / 1000, 'uint32');
red = cast((RRRGGGBBB - (green * 1000) - blue) / 1000000, 'uint32');

RRGGBBAA = bitshift(red, 16) + bitshift(green, 8) + blue;
